simulink model "DTNPC_Inverter"  (R2023b)
settings: Solver=VariableStepAuto  StartTime=0.0  StopTime=1  RelTol=1e-3
libraries: spsSeriesRLCBranchLib x13, spsIGBTDiodeLib x8, spsIGBTLib x6, spsVoltageMeasurementLib x6, spsCurrentMeasurementLib x3, spsRMSLib x2, spsDCVoltageSourceLib x1, simulink x1, spsMeanLib x1, spsTHDLib x1, spspowerguiLib x1
settings Model: SimulationMode=accelerator  Creator=abc6820292  LastModifiedBy=Qu
settings DebuggingCC: UnconnectedInputMsg=warning  UnconnectedOutputMsg=warning  UnconnectedLineMsg=warning
settings ModelReferenceCC: EnableRefExpFcnMdlSchedulingChecks=on
settings RTWCC: DLArmComputeVersion=19.05

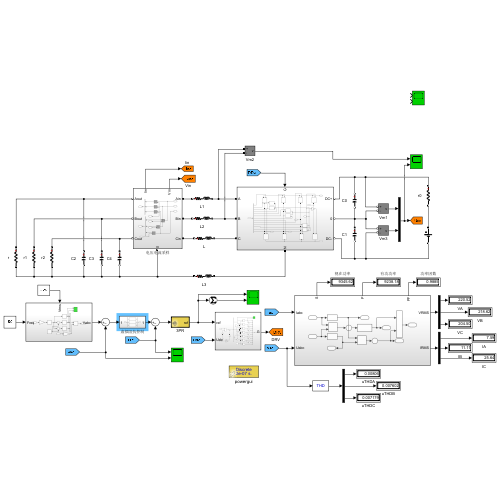
[thumbnail: Simulink's stored preview of the top-level diagram]
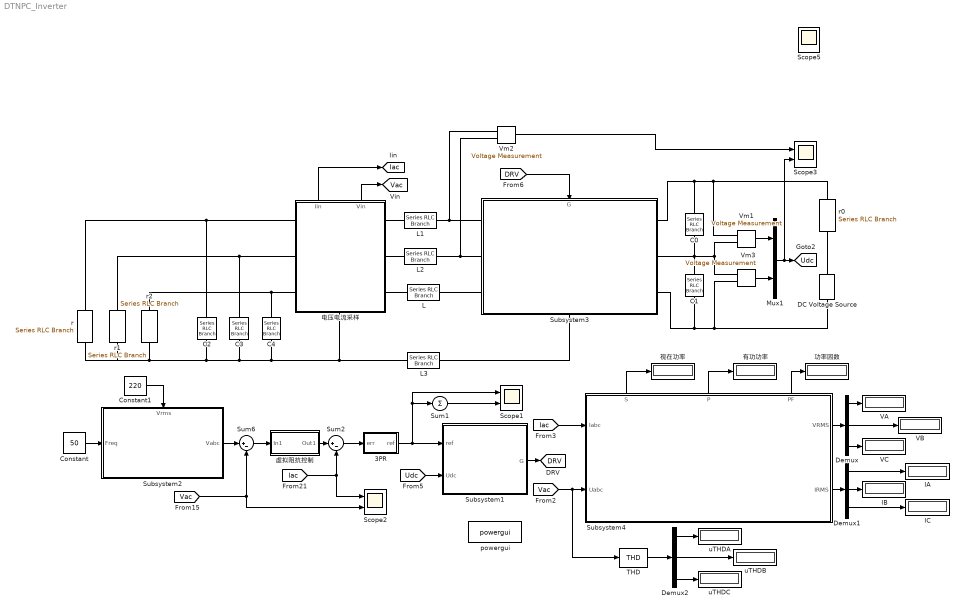
== system DTNPC_Inverter ==
  3PR : Subsystem  TreatAsAtomicUnit=on  mask{Kp=4, Kr=100, Wc=5, Upper=400, Lower=-400}
  C0 : spsSeriesRLCBranchLib/Series RLC Branch  LConnTagsString=__new0  RConnTagsString=__new0  BranchType=C  Resistance=0  Inductance=0  SetiL0=off  InitialCurrent=0  Capacitance=2e-3  Setx0=on  InitialVoltage=350  Measurements=None
  C1 : spsSeriesRLCBranchLib/Series RLC Branch  LConnTagsString=__new0  RConnTagsString=__new0  BranchType=C  Resistance=0  Inductance=0  SetiL0=off  InitialCurrent=0  Capacitance=2e-3  Setx0=on  InitialVoltage=350  Measurements=None
  C2 : spsSeriesRLCBranchLib/Series RLC Branch  LConnTagsString=__new0  RConnTagsString=__new0  BranchType=C  Resistance=0  Inductance=0  SetiL0=off  InitialCurrent=0  Capacitance=1e-5  Setx0=off  InitialVoltage=310  Measurements=None
  C3 : spsSeriesRLCBranchLib/Series RLC Branch  LConnTagsString=__new0  RConnTagsString=__new0  BranchType=C  Resistance=0  Inductance=0  SetiL0=off  InitialCurrent=0  Capacitance=1e-5  Setx0=off  InitialVoltage=310  Measurements=None
  C4 : spsSeriesRLCBranchLib/Series RLC Branch  LConnTagsString=__new0  RConnTagsString=__new0  BranchType=C  Resistance=0  Inductance=0  SetiL0=off  InitialCurrent=0  Capacitance=1e-5  Setx0=off  InitialVoltage=310  Measurements=None
  Constant : Constant  Value=50
  Constant1 : Constant  Value=220
  DC Voltage Source : spsDCVoltageSourceLib/DC Voltage Source  Amplitude=700  Measurements=None
  Demux : Demux  Outputs=3
  Demux1 : Demux  Outputs=3
  Demux2 : Demux  Outputs=3
  IA : Display
      settings: Format=bank
  IB : Display
      settings: Format=bank
  IC : Display
      settings: Format=bank
  L : spsSeriesRLCBranchLib/Series RLC Branch  LConnTagsString=__new0  RConnTagsString=__new0  BranchType=RL  Resistance=1  Inductance=5e-4  SetiL0=off  InitialCurrent=0  Capacitance=inf  Setx0=off  InitialVoltage=0  Measurements=None
  L1 : spsSeriesRLCBranchLib/Series RLC Branch  LConnTagsString=__new0  RConnTagsString=__new0  BranchType=RL  Resistance=1  Inductance=5e-4  SetiL0=off  InitialCurrent=0  Capacitance=inf  Setx0=off  InitialVoltage=0  Measurements=None
  L2 : spsSeriesRLCBranchLib/Series RLC Branch  LConnTagsString=__new0  RConnTagsString=__new0  BranchType=RL  Resistance=1  Inductance=5e-4  SetiL0=off  InitialCurrent=0  Capacitance=inf  Setx0=off  InitialVoltage=0  Measurements=None
  L3 : spsSeriesRLCBranchLib/Series RLC Branch  LConnTagsString=__new0  RConnTagsString=__new0  BranchType=RL  Resistance=0.01  Inductance=2e-4  SetiL0=off  InitialCurrent=0  Capacitance=inf  Setx0=off  InitialVoltage=0  Measurements=None
  Mux1 : Mux  Inputs=2
  Scope{1..3,5} (4 alike) : Scope  NumInputPorts=2
  Subsystem1 : Subsystem
  Subsystem2 : Subsystem
      settings: PortSchema="{\"entries\":[{\"content\":{\"sides\":[{\"content\":{\"connectorIds\":[\"In1\"]},\"type\":\"ConnectorPlacement.EquallySpacedRectSide\",\"uuid\":\"b83f0250-9c61-4256-afad-581095ab140f\"},{\"content\":{\"connectorIds\":[\"Out1\"],\"side\":\"RIGHT\"},\"type\":\"ConnectorPlacement.EquallySpacedRectSide\",\"uuid\":\"e21d95d9-bd65-4b8b-8e7b-d6ad7b8ad5cc\"},{\"content\":{\"connectorIds\":[\"In2\"],\"side\":\"TOP\"},\"type\":\"ConnectorPlacement.EquallySpacedRectSide\",\"uuid\":\"3e84556d-e7a5-4296-98ac-10e766fe76c2\"}]},\"type\":\"ConnectorPlacement.EquallySpacedConnector\",\"uuid\":\"d357bca2-f059-42e0-868e-69ff40dc2149\"}],\"packageUris\":[\"http://schema.mathworks.com/mf0/Connector/R2020b\"],\"version\":\"1.0\"}"
  Subsystem3 : Subsystem
      settings: PortSchema="{\"entries\":[{\"content\":{\"sides\":[{\"content\":{\"connectorIds\":[\"LConn1\",\"LConn2\",\"LConn3\"]},\"type\":\"ConnectorPlacement.EquallySpacedRectSide\",\"uuid\":\"78b2e702-d06c-4e88-88fa-76d063fe9b62\"},{\"content\":{\"connectorIds\":[\"RConn1\",\"RConn2\",\"RConn3\"],\"side\":\"RIGHT\"},\"type\":\"ConnectorPlacement.EquallySpacedRectSide\",\"uuid\":\"7bc0c85a-fd6f-4f5e-acb5-d7baabe65af7\"},{\"content\":{\"connectorIds\":[\"In1\"],\"side\":\"TOP\"},\"type\":\"ConnectorPlacement.EquallySpacedRectSide\",\"uuid\":\"08102ab6-f4c4-4a42-9468-f733ccd64290\"},{\"content\":{\"connectorIds\":[\"RConn4\"],\"side\":\"BOTTOM\"},\"type\":\"ConnectorPlacement.EquallySpacedRectSide\",\"uuid\":\"d24dfa10-9dd8-43ca-ac07-c82c5936d107\"}]},\"type\":\"ConnectorPlacement.EquallySpacedConnector\",\"uuid\":\"9f42a9a1-5471-4f27-a0ba-eb296522cfc6\"}],\"packageUris\":[\"http://schema.mathworks.com/mf0/Connector/R2020b\"],\"version\":\"1.0\"}"
  Subsystem4 : Subsystem
      settings: PortSchema="{\"entries\":[{\"content\":{\"sides\":[{\"content\":{\"connectorIds\":[\"In1\",\"In2\"]},\"type\":\"ConnectorPlacement.EquallySpacedRectSide\",\"uuid\":\"8f3b7bf1-7c44-4492-a357-aa6e3e6d66a4\"},{\"content\":{\"connectorIds\":[\"Out1\",\"Out2\"],\"side\":\"RIGHT\"},\"type\":\"ConnectorPlacement.EquallySpacedRectSide\",\"uuid\":\"7ae784cf-6bcf-4684-9c07-1770fc60c8a0\"},{\"content\":{\"connectorIds\":[\"Out3\",\"Out4\",\"Out5\"],\"side\":\"TOP\"},\"type\":\"ConnectorPlacement.EquallySpacedRectSide\",\"uuid\":\"0e016931-6232-4ad6-afe9-572a0571336f\"},{\"content\":{\"side\":\"BOTTOM\"},\"type\":\"ConnectorPlacement.EquallySpacedRectSide\",\"uuid\":\"ef67c6ee-ba81-4705-af34-81581e7e9907\"}]},\"type\":\"ConnectorPlacement.EquallySpacedConnector\",\"uuid\":\"922af512-c0ff-443f-816c-194775a78dc8\"}],\"packageUris\":[\"http://schema.mathworks.com/mf0/Connector/R2020b\"],\"version\":\"1.0\"}"
  Sum1 : Sum  Inputs=+
  Sum2 : Sum  Inputs=|+-
  Sum6 : Sum  Inputs=|+-
  THD : spsTHDLib/THD  Freq=50  Ts=0
  VA : Display
      settings: Format=bank
  VB : Display
      settings: Format=bank
  VC : Display
      settings: Format=bank
  Vm1 : spsVoltageMeasurementLib/Voltage Measurement  PhasorSimulation=off  OutputType=Complex  PSBequivalent=0
  Vm2 : spsVoltageMeasurementLib/Voltage Measurement  PhasorSimulation=off  OutputType=Complex  PSBequivalent=0
  Vm3 : spsVoltageMeasurementLib/Voltage Measurement  PhasorSimulation=off  OutputType=Complex  PSBequivalent=0
  powergui : spspowerguiLib/powergui  SimulationMode=Discrete  SampleTime=2e-7  frequency=60  Iterations=50  frequencyindice=0  Pbase=100e6  ErrMax=1e-4  UnitsV=kV  UnitsW=MW  buscounter=0  FunctionMessages=off  echomessages=off  EnableUseOfTLC=off  CurrentSourceSwitches=off  DisableSnubberDevices=off  DisableRonSwitches=off  DisableVfSwitches=off  DisplayEquations=off  AutomaticDiscreteSolvers=off  SolverType=Tustin/Backward Euler (TBE)  Interpol=off  ExternalGateDelay=off  methode=off  Ts=0  x0status=blocks  SPID=off  SwTol=0  HookPort=off  NonlinearTolerance=1e-4  nMaxIteration=100  ContinueOnMaxIteration=off  RestoreLinks=warning  ResistiveCurrentMeasurement=off  Frange=[0:2:500]  Ylog=off  Xlog=on  ShowGrid=off  save=off  variable=ZData  structure=QQQQQ  ZoomFFT=off  StartTime=0.5  cycles=15  DisplayStyle=1  fundamental=50  FreqAxis=off  MaxFrequency=1000  frequencyindicesteady=1  RmsSteady=1  display=off
  r : spsSeriesRLCBranchLib/Series RLC Branch  LConnTagsString=__new0  RConnTagsString=__new0  BranchType=R  Resistance=30  Inductance=12e-4  SetiL0=off  InitialCurrent=0  Capacitance=inf  Setx0=off  InitialVoltage=0  Measurements=None
  r0 : spsSeriesRLCBranchLib/Series RLC Branch  LConnTagsString=__new0  RConnTagsString=__new0  BranchType=R  Resistance=0.1  Inductance=12e-4  SetiL0=off  InitialCurrent=0  Capacitance=inf  Setx0=off  InitialVoltage=0  Measurements=None
  r1 : spsSeriesRLCBranchLib/Series RLC Branch  LConnTagsString=__new0  RConnTagsString=__new0  BranchType=R  Resistance=20  Inductance=12e-4  SetiL0=off  InitialCurrent=0  Capacitance=inf  Setx0=off  InitialVoltage=0  Measurements=None
  r2 : spsSeriesRLCBranchLib/Series RLC Branch  LConnTagsString=__new0  RConnTagsString=__new0  BranchType=R  Resistance=8  Inductance=12e-4  SetiL0=off  InitialCurrent=0  Capacitance=inf  Setx0=off  InitialVoltage=0  Measurements=None
  uTHDA : Display
  uTHDB : Display
  uTHDC : Display
  功率因数 : Display
  有功功率 : Display
      settings: Format=bank
  电压电流采样 : Subsystem
      settings: PortSchema="{\"entries\":[{\"content\":{\"sides\":[{\"content\":{\"connectorIds\":[\"LConn1\",\"LConn2\",\"LConn3\"]},\"type\":\"ConnectorPlacement.EquallySpacedRectSide\",\"uuid\":\"d60dd16a-7a74-435a-96f5-79c0993f3801\"},{\"content\":{\"connectorIds\":[\"RConn1\",\"RConn2\",\"RConn3\"],\"side\":\"RIGHT\"},\"type\":\"ConnectorPlacement.EquallySpacedRectSide\",\"uuid\":\"38a0d536-50a5-43bd-9d58-6b0db9c378a0\"},{\"content\":{\"connectorIds\":[\"Out1\",\"Out2\"],\"side\":\"TOP\"},\"type\":\"ConnectorPlacement.EquallySpacedRectSide\",\"uuid\":\"65be575f-dbb8-4f94-beb1-b426df65c1d5\"},{\"content\":{\"connectorIds\":[\"RConn4\"],\"side\":\"BOTTOM\"},\"type\":\"ConnectorPlacement.EquallySpacedRectSide\",\"uuid\":\"a28dffe8-15db-4523-b673-2414d0fbe1e1\"}]},\"type\":\"ConnectorPlacement.EquallySpacedConnector\",\"uuid\":\"1fc3ca7a-50b1-4fd5-a5d3-d39cc1e6f07d\"}],\"packageUris\":[\"http://schema.mathworks.com/mf0/Connector/R2020b\"],\"version\":\"1.0\"}"
  虚拟阻抗控制 : Subsystem
  视在功率 : Display
      settings: Format=bank
  tag scope: DRV=global, Iac=global, Udc=global, Vac=global
  wires:
  Vm2/1 -> Scope3/1
  [Udc] -> Subsystem1/2(Udc)
  3PR/1(ref) -> Sum1/1, Scope1/1, Subsystem1/1(ref)
  Subsystem4/5(PF) -> 功率因数/1
  THD/1 -> Demux2/1
  Subsystem4/4(P) -> 有功功率/1
  电压电流采样/2(Iin) -> [Iac]
  Demux/3 -> VC/1
  Subsystem4/2(IRMS) -> Demux1/1
  Demux2/1 -> uTHDA/1
  [Iac] -> Subsystem4/1(Iabc)
  Subsystem4/1(VRMS) -> Demux/1
  Demux/1 -> VA/1
  Demux/2 -> VB/1
  Demux1/1 -> IA/1
  Demux1/2 -> IB/1
  Demux2/2 -> uTHDB/1
  Demux1/3 -> IC/1
  Demux2/3 -> uTHDC/1
  电压电流采样/1(Vin) -> [Vac]
  Vm3/1 -> Mux1/2
  [Vac] -> Sum6/2, Scope2/2
  Vm1/1 -> Mux1/1
  Mux1/1 -> Scope3/2, [Udc]
  Sum2/1 -> 3PR/1(err)
  [Iac] -> Sum2/2, Scope2/1
  Subsystem1/1(G) -> [DRV]
  虚拟阻抗控制/1(Out1) -> Sum2/1
  Sum6/1 -> 虚拟阻抗控制/1(In1)
  Subsystem2/1(Vabc) -> Sum6/1
  Constant/1 -> Subsystem2/1(Freq)
  Constant1/1 -> Subsystem2/2(Vrms)
  Sum1/1 -> Scope1/2
  [DRV] -> Subsystem3/1(G)
  [Vac] -> THD/1, Subsystem4/2(Uabc)
  Subsystem4/3(S) -> 视在功率/1
  connections:
  C1/RConn1 -- Subsystem3/RConn3 -- DC Voltage Source/LConn1 -- Vm3/LConn2
  C0/LConn1 -- Subsystem3/RConn1 -- r0/LConn1 -- Vm1/LConn1
  L/RConn1 -- Subsystem3/LConn3
  L2/RConn1 -- Vm2/LConn2 -- Subsystem3/LConn2
  L1/RConn1 -- Vm2/LConn1 -- Subsystem3/LConn1
  电压电流采样/LConn1 -- L1/LConn1
  电压电流采样/LConn2 -- L2/LConn1
  电压电流采样/LConn3 -- L/LConn1
  C4/LConn1 -- r2/LConn1 -- 电压电流采样/RConn3
  C3/LConn1 -- r1/LConn1 -- 电压电流采样/RConn2
  C2/LConn1 -- r/LConn1 -- 电压电流采样/RConn1
  DC Voltage Source/RConn1 -- r0/RConn1
  Vm3/LConn1 -- Subsystem3/RConn2 -- C0/RConn1 -- C1/LConn1 -- Vm1/LConn2
  C3/RConn1 -- r1/RConn1 -- r/RConn1 -- r2/RConn1 -- C2/RConn1 -- C4/RConn1 -- 电压电流采样/RConn4 -- L3/LConn1
  L3/RConn1 -- Subsystem3/RConn4

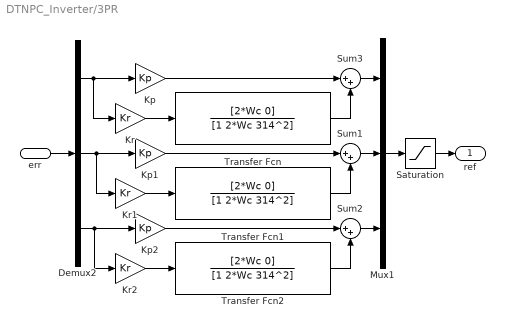
== system DTNPC_Inverter/3PR ==
  err : Inport
  Demux2 : Demux  Outputs=3
  Kp : Gain  Gain=Kp
  Kp1 : Gain  Gain=Kp
  Kp2 : Gain  Gain=Kp
  Kr : Gain  Gain=Kr
  Kr1 : Gain  Gain=Kr
  Kr2 : Gain  Gain=Kr
  Mux1 : Mux  Inputs=3
  Saturation : Saturate  UpperLimit=Upper  LowerLimit=Lower
  Sum1 : Sum  Inputs=|++
  Sum2 : Sum  Inputs=|++
  Sum3 : Sum  Inputs=|++
  Transfer Fcn : TransferFcn  Numerator=[2*Wc 0]  Denominator=[1 2*Wc 314^2]
  Transfer Fcn1 : TransferFcn  Numerator=[2*Wc 0]  Denominator=[1 2*Wc 314^2]
  Transfer Fcn2 : TransferFcn  Numerator=[2*Wc 0]  Denominator=[1 2*Wc 314^2]
  ref : Outport
  wires:
  Kp/1 -> Sum3/1
  err/1 -> Demux2/1
  Kr/1 -> Transfer Fcn/1
  Transfer Fcn/1 -> Sum3/2
  Saturation/1 -> ref/1
  Sum3/1 -> Mux1/1
  Kr1/1 -> Transfer Fcn1/1
  Kp1/1 -> Sum1/1
  Transfer Fcn1/1 -> Sum1/2
  Sum1/1 -> Mux1/2
  Kr2/1 -> Transfer Fcn2/1
  Kp2/1 -> Sum2/1
  Transfer Fcn2/1 -> Sum2/2
  Sum2/1 -> Mux1/3
  Mux1/1 -> Saturation/1
  Demux2/1 -> Kr/1, Kp/1
  Demux2/2 -> Kr1/1, Kp1/1
  Demux2/3 -> Kr2/1, Kp2/1

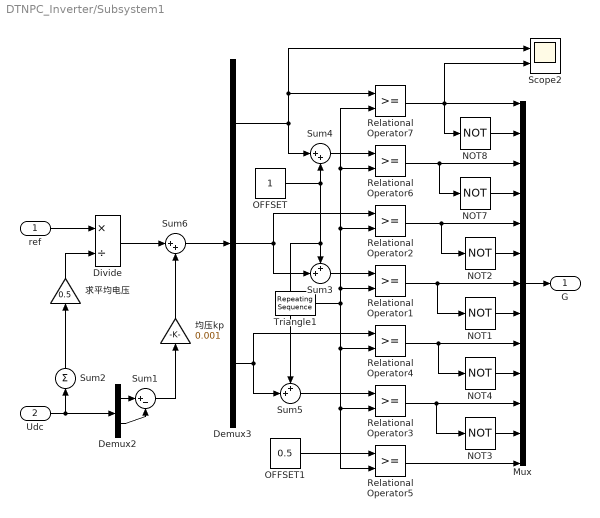
== system DTNPC_Inverter/Subsystem1 ==
  ref : Inport
  Udc : Inport  Port=2
  Demux2 : Demux  Outputs=2
  Demux3 : Demux  Outputs=3
  Divide : Product  Inputs=*/
  Mux : Mux  Inputs=13
  NOT{1..4,7..8} (6 alike) : Logic  Operator=NOT  IconShape=distinctive  AllPortsSameDT=off  OutDataTypeStr=boolean
  OFFSET : Constant
  OFFSET1 : Constant  Value=0.5
  Relational Operator{1..7} (7 alike) : RelationalOperator  OutDataTypeStr=boolean  InputSameDT=off
  Scope2 : Scope  NumInputPorts=2
  Sum1 : Sum  Inputs=|+-
  Sum2 : Sum  Inputs=+
  Sum3 : Sum  Inputs=++|
  Sum4 : Sum  Inputs=|++
  Sum5 : Sum  Inputs=++|
  Sum6 : Sum  Inputs=|++
  Triangle1 : simulink/Sources/Repeating Sequence  rep_seq_t=[0 1/20000/2 1/20000]  rep_seq_y=[0 1 0]
  均压kp : Gain  Gain=0.001
  求平均电压 : Gain  Gain=0.5
  G : Outport
  wires:
  ref/1 -> Divide/1
  Demux2/1 -> Sum1/1
  Demux2/2 -> Sum1/2
  Sum1/1 -> 均压kp/1
  Udc/1 -> Demux2/1, Sum2/1
  Divide/1 -> Sum6/1
  求平均电压/1 -> Divide/2
  Sum2/1 -> 求平均电压/1
  Relational Operator6/1 -> NOT7/1, Mux/3
  Sum3/1 -> Relational Operator1/1
  Sum5/1 -> Relational Operator3/1
  Sum4/1 -> Relational Operator6/1
  Relational Operator1/1 -> Mux/7, NOT1/1
  Relational Operator3/1 -> NOT3/1, Mux/11
  NOT7/1 -> Mux/4
  Sum6/1 -> Demux3/1
  Demux3/1 -> Sum4/1, Scope2/1, Relational Operator7/1
  Relational Operator4/1 -> Mux/9, NOT4/1
  NOT1/1 -> Mux/8
  Demux3/2 -> Relational Operator2/1, Sum3/2
  Relational Operator2/1 -> Mux/5, NOT2/1
  OFFSET/1 -> Sum5/1, Sum3/1, Sum4/2
  NOT3/1 -> Mux/12
  Triangle1/1 -> Relational Operator5/2, Relational Operator3/2, Relational Operator4/2, Relational Operator1/2, Relational Operator2/2, Relational Operator7/2, Relational Operator6/2
  Demux3/3 -> Relational Operator4/1, Sum5/2
  Relational Operator7/1 -> Scope2/2, Mux/1, NOT8/1
  Mux/1 -> G/1
  NOT4/1 -> Mux/10
  NOT2/1 -> Mux/6
  NOT8/1 -> Mux/2
  Relational Operator5/1 -> Mux/13
  OFFSET1/1 -> Relational Operator5/1
  均压kp/1 -> Sum6/2

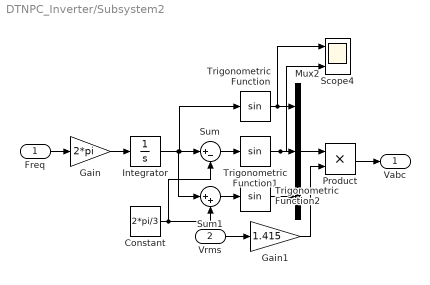
== system DTNPC_Inverter/Subsystem2 ==
  Freq : Inport
  Vrms : Inport  Port=2
  Constant : Constant  Value=2*pi/3
  Gain : Gain  Gain=2*pi
  Gain1 : Gain  Gain=1.415
  Integrator : Integrator  WrapState=on  WrappedStateUpperValue=2*pi  WrappedStateLowerValue=0
  Mux2 : Mux  Inputs=3
  Product : Product
  Scope4 : Scope  NumInputPorts=2
  Sum : Sum  Inputs=|+-
  Sum1 : Sum  Inputs=|++
  Trigonometric Function : Trigonometry
  Trigonometric Function1 : Trigonometry
  Trigonometric Function2 : Trigonometry
  Vabc : Outport
  wires:
  Gain/1 -> Integrator/1
  Freq/1 -> Gain/1
  Integrator/1 -> Sum1/1, Trigonometric Function/1, Sum/1
  Constant/1 -> Sum1/2, Sum/2
  Sum/1 -> Trigonometric Function1/1
  Sum1/1 -> Trigonometric Function2/1
  Trigonometric Function/1 -> Scope4/1, Mux2/1
  Trigonometric Function1/1 -> Scope4/2, Mux2/2
  Trigonometric Function2/1 -> Mux2/3
  Mux2/1 -> Product/1
  Product/1 -> Vabc/1
  Vrms/1 -> Gain1/1
  Gain1/1 -> Product/2

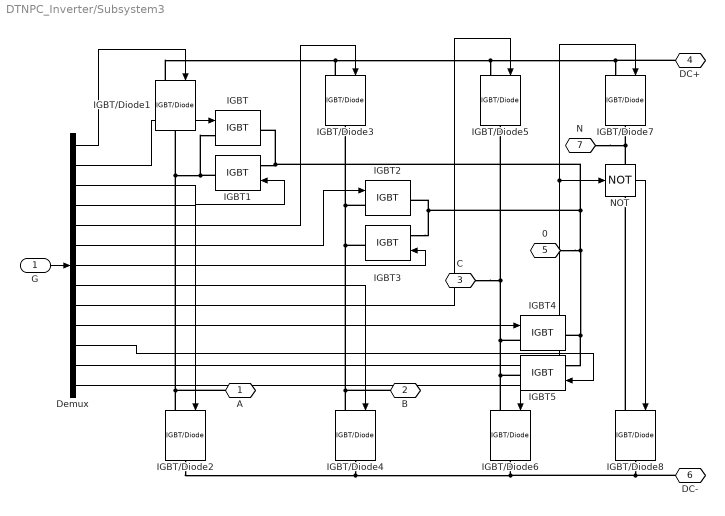
== system DTNPC_Inverter/Subsystem3 ==
  G : Inport
  Demux : Demux  Outputs=13
  IGBT{,1..5} (6 alike) : spsIGBTLib/IGBT  Ron=0.001  Lon=0  Vf=1  Tf=1e-6  Tt=2e-6  IC=0  Rs=1e5  Cs=inf  Measurements=off
  IGBT/Diode{1..8} (8 alike) : spsIGBTDiodeLib/IGBT//Diode  Ron=1e-3  Rs=1e5  Cs=inf  Measurements=off
  NOT : Logic  Operator=NOT  IconShape=distinctive  AllPortsSameDT=off  OutDataTypeStr=boolean
  A : PMIOPort  Side=Left
  B : PMIOPort  Port=2  Side=Left
  C : PMIOPort  Port=3  Side=Left
  DC+ : PMIOPort  Port=4  Side=Right
  0 : PMIOPort  Port=5  Side=Right
  DC- : PMIOPort  Port=6  Side=Right
  N : PMIOPort  Port=7  Side=Right
  wires:
  G/1 -> Demux/1
  Demux/1 -> IGBT/Diode1/1
  Demux/4 -> IGBT/Diode2/1
  Demux/2 -> IGBT/1
  Demux/3 -> IGBT1/1
  Demux/5 -> IGBT/Diode3/1
  Demux/8 -> IGBT/Diode4/1
  Demux/6 -> IGBT2/1
  Demux/7 -> IGBT3/1
  Demux/12 -> IGBT/Diode6/1
  Demux/9 -> IGBT/Diode5/1
  Demux/10 -> IGBT4/1
  Demux/11 -> IGBT5/1
  Demux/13 -> NOT/1, IGBT/Diode7/1
  NOT/1 -> IGBT/Diode8/1
  connections:
  A/RConn1 -- IGBT/Diode2/LConn1 -- IGBT/Diode1/RConn1 -- IGBT/LConn1 -- IGBT1/RConn1
  IGBT5/LConn1 -- IGBT2/RConn1 -- IGBT3/LConn1 -- IGBT/RConn1 -- IGBT1/LConn1 -- 0/RConn1 -- IGBT4/RConn1
  IGBT/Diode4/LConn1 -- B/RConn1 -- IGBT3/RConn1 -- IGBT2/LConn1 -- IGBT/Diode3/RConn1
  IGBT/Diode6/LConn1 -- C/RConn1 -- IGBT/Diode5/RConn1 -- IGBT4/LConn1 -- IGBT5/RConn1
  IGBT/Diode2/RConn1 -- IGBT/Diode4/RConn1 -- DC-/RConn1 -- IGBT/Diode8/RConn1 -- IGBT/Diode6/RConn1
  IGBT/Diode8/LConn1 -- N/RConn1 -- IGBT/Diode7/RConn1
  IGBT/Diode1/LConn1 -- IGBT/Diode3/LConn1 -- IGBT/Diode7/LConn1 -- DC+/RConn1 -- IGBT/Diode5/LConn1

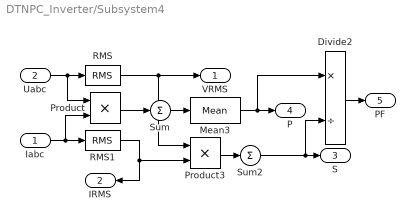
== system DTNPC_Inverter/Subsystem4 ==
  Iabc : Inport
  Uabc : Inport  Port=2
  Divide2 : Product  Inputs=*/
  Mean3 : spsMeanLib/Mean  Freq=50  Vinit=0  Ts=0
  Product : Product
  Product3 : Product
  RMS : spsRMSLib/RMS  TrueRMS=on  Freq=50  RMSInit=0  Ts=0
  RMS1 : spsRMSLib/RMS  TrueRMS=on  Freq=50  RMSInit=0  Ts=0
  Sum : Sum  Inputs=+
  Sum2 : Sum  Inputs=+
  VRMS : Outport
  IRMS : Outport  Port=2
  S : Outport  Port=3
  P : Outport  Port=4
  PF : Outport  Port=5
  wires:
  Iabc/1 -> Product/2, RMS1/1
  RMS/1 -> VRMS/1, Product3/1
  RMS1/1 -> Product3/2, IRMS/1
  Divide2/1 -> PF/1
  Mean3/1 -> Divide2/1, P/1
  Sum/1 -> Mean3/1
  Uabc/1 -> RMS/1, Product/1
  Product/1 -> Sum/1
  Product3/1 -> Sum2/1
  Sum2/1 -> Divide2/2, S/1

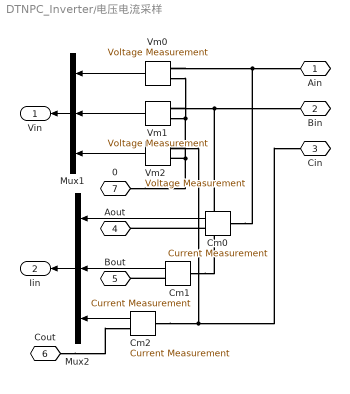
== system DTNPC_Inverter/电压电流采样 ==
  Cm0 : spsCurrentMeasurementLib/Current Measurement  PhasorSimulation=off  OutputType=Complex  PSBequivalent=0
  Cm1 : spsCurrentMeasurementLib/Current Measurement  PhasorSimulation=off  OutputType=Complex  PSBequivalent=0
  Cm2 : spsCurrentMeasurementLib/Current Measurement  PhasorSimulation=off  OutputType=Complex  PSBequivalent=0
  Mux1 : Mux  Inputs=3
  Mux2 : Mux  Inputs=3
  Vm0 : spsVoltageMeasurementLib/Voltage Measurement  PhasorSimulation=off  OutputType=Complex  PSBequivalent=0
  Vm1 : spsVoltageMeasurementLib/Voltage Measurement  PhasorSimulation=off  OutputType=Complex  PSBequivalent=0
  Vm2 : spsVoltageMeasurementLib/Voltage Measurement  PhasorSimulation=off  OutputType=Complex  PSBequivalent=0
  Ain : PMIOPort  Side=Left
  Bin : PMIOPort  Port=2  Side=Left
  Cin : PMIOPort  Port=3  Side=Left
  Aout : PMIOPort  Port=4  Side=Right
  Bout : PMIOPort  Port=5  Side=Right
  Cout : PMIOPort  Port=6  Side=Right
  0 : PMIOPort  Port=7  Side=Right
  Vin : Outport
  Iin : Outport  Port=2
  wires:
  Cm2/1 -> Mux2/3
  Vm1/1 -> Mux1/2
  Cm1/1 -> Mux2/2
  Vm2/1 -> Mux1/3
  Vm0/1 -> Mux1/1
  Mux1/1 -> Vin/1
  Cm0/1 -> Mux2/1
  Mux2/1 -> Iin/1
  connections:
  Vm1/LConn1 -- Cm1/LConn1 -- Bin/RConn1
  Cm0/RConn1 -- Aout/RConn1
  Vm0/LConn1 -- Cm0/LConn1 -- Ain/RConn1
  Cm2/LConn1 -- Vm2/LConn1 -- Cin/RConn1
  Cm1/RConn1 -- Bout/RConn1
  Cout/RConn1 -- Cm2/RConn1
  0/RConn1 -- Vm0/LConn2 -- Vm1/LConn2 -- Vm2/LConn2

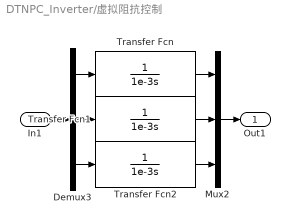
== system DTNPC_Inverter/虚拟阻抗控制 ==
  In1 : Inport
  Demux3 : Demux  Outputs=3
  Mux2 : Mux  Inputs=3
  Transfer Fcn : TransferFcn  Denominator=[1e-3 0]
  Transfer Fcn1 : TransferFcn  Denominator=[1e-3 0]
  Transfer Fcn2 : TransferFcn  Denominator=[1e-3 0]
  Out1 : Outport
  wires:
  Demux3/2 -> Transfer Fcn1/1
  Transfer Fcn/1 -> Mux2/1
  Mux2/1 -> Out1/1
  Transfer Fcn1/1 -> Mux2/2
  Transfer Fcn2/1 -> Mux2/3
  Demux3/3 -> Transfer Fcn2/1
  Demux3/1 -> Transfer Fcn/1
  In1/1 -> Demux3/1
